simulink model "test_thrust"  (R2024b)
settings: Solver=FixedStepAuto  StartTime=0.0  StopTime=inf  FixedStep=0.01  RelTol=1e-3  EnableMultiTasking=on
libraries: px4Sensorslib x3, px4Peripheralslib x1
settings Model: SimulationMode=external  ExtModeTrigDuration=10  Creator=ArriGE66  LastModifiedBy=xippa
settings SolverCC: PositivePriorityOrder=on
settings OptimizationCC: EnhancedBackFolding=on  PassReuseOutputArgsAs=Individual arguments  ZeroExternalMemoryAtStartup=off  ZeroInternalMemoryAtStartup=off  MaxStackSize=64  OptimizeBlockOrder=speed  DifferentSizesBufferReuse=on  OptimizationCustomize=off  EfficientTunableParamExpr=on
settings DebuggingCC: ParameterTunabilityLossMsg=error
settings HardwareCC: ProdBitPerPointer=32  ProdBitPerSizeT=32  ProdBitPerPtrDiffT=32  ProdLargestAtomicInteger=Long  ProdLargestAtomicFloat=Double  ProdWordSize=32  ProdLongLongMode=on  ProdHWDeviceType=ARM Compatible->ARM Cortex
settings SFSimCC: MATLABDynamicMemAlloc=off  SimTargetLang=C++
settings RTWCC: Description=Embedded Coder  SystemTargetFile=ert.tlc  HardwareBoard=PX4 Cube Orange  TemplateMakefile=ert_default_tmf  Toolchain=GNU Tools for PX4 Autopilots  TargetLang=C++  GPUComputeCapability=3.5
settings CodeAppCC: ForceParamTrailComments=on  IgnoreCustomStorageClasses=off  OperatorAnnotations=on  SimulinkDataObjDesc=on  SFDataObjDesc=on  InsertBlockDesc=on
settings ERTTargetCC: ExtMode=on  ExtModeTransport=3  ExtModeStaticAlloc=on  ExtModeStaticAllocSize=1024  ExtModeMexFile=ext_xcp  ExtModeMexArgs=1 COM10 3000000  ExtModeIntrfLevel=Level2 - Open  InlinedParameterPlacement=Hierarchical  DynamicArrayContainerType=coder::array

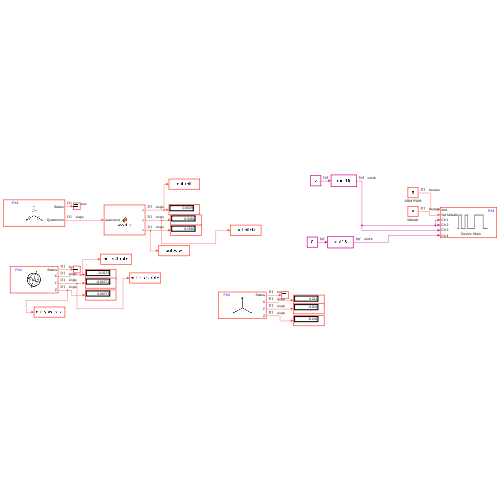
[thumbnail: Simulink's stored preview of the top-level diagram]
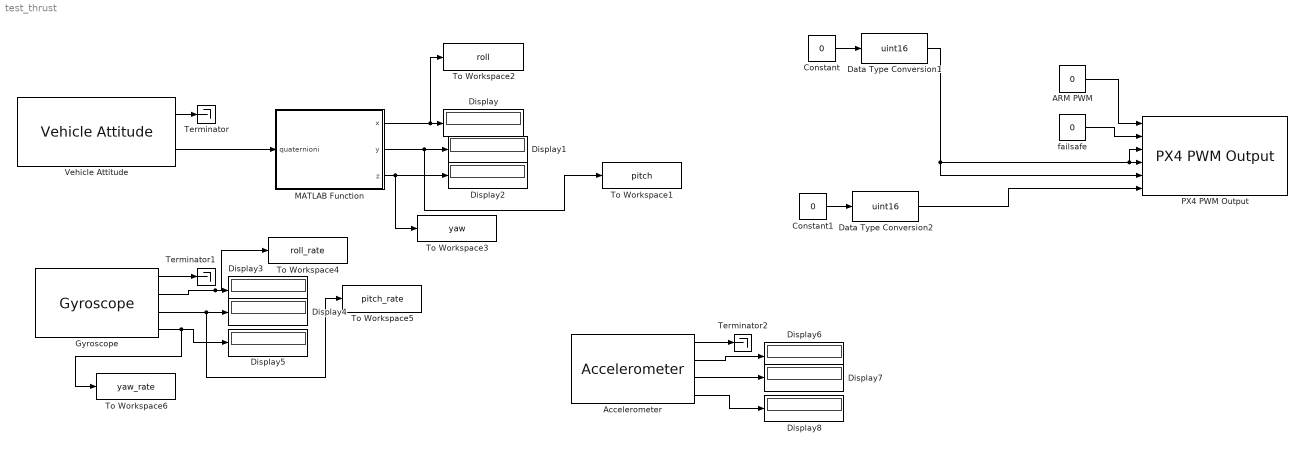
== system test_thrust ==
  ARM PWM : Constant  Value=0  OutDataTypeStr=boolean  SampleTime=1/100
  Accelerometer : px4Sensorslib/Accelerometer  uorbTimeStamp=off  BlockingMode=off  BlockTimeout=1e-3  sampleTime=1/100
  Constant : Constant  Value=0
  Constant1 : Constant  Value=0
  Data Type Conversion1 : DataTypeConversion  OutDataTypeStr=uint16  SaturateOnIntegerOverflow=off  RndMeth=Floor
  Data Type Conversion2 : DataTypeConversion  OutDataTypeStr=uint16  SaturateOnIntegerOverflow=off  RndMeth=Floor
  Display{,1..8} (9 alike) : Display
  Gyroscope : px4Sensorslib/Gyroscope  uorbTimeStamp=off  BlockingMode=off  BlockTimeout=1e-3  sampleTime=1/100
  MATLAB Function : MATLAB Function  TreatAsAtomicUnit=on
  PX4 PWM Output : px4Peripheralslib/PX4 PWM Output  pwmDevice=Main  pwmChannel1_=on  pwmChannel2_=on  pwmChannel3_=on  pwmChannel4_=on  pwmChannel5_=off  pwmChannel6_=off  pwmChannel7_=off  pwmChannel8_=off
  Terminator : Terminator
  Terminator1 : Terminator
  Terminator2 : Terminator
  To Workspace1 : ToWorkspace  VariableName=pitch  SaveFormat=Timeseries  SampleTime=-1
  To Workspace2 : ToWorkspace  VariableName=roll  SaveFormat=Timeseries  SampleTime=-1
  To Workspace3 : ToWorkspace  VariableName=yaw  SaveFormat=Timeseries  SampleTime=-1
  To Workspace4 : ToWorkspace  VariableName=roll_rate  SaveFormat=Timeseries  SampleTime=-1
  To Workspace5 : ToWorkspace  VariableName=pitch_rate  SaveFormat=Timeseries  SampleTime=-1
  To Workspace6 : ToWorkspace  VariableName=yaw_rate  SaveFormat=Timeseries  SampleTime=-1
  Vehicle Attitude : px4Sensorslib/Vehicle Attitude  rollRate=off  pitchRate=off  yawRate=off  quaternion=on  uorbTimeStamp=off  BlockingMode=off  BlockTimeout=0.001  sampleTime=1/100
  failsafe : Constant  Value=0  OutDataTypeStr=boolean  SampleTime=0.01
  wires:
  Vehicle Attitude/2 -> MATLAB Function/1(quaternioni)
  Vehicle Attitude/1 -> Terminator/1
  Data Type Conversion1/1 -> PX4 PWM Output/3, PX4 PWM Output/4, PX4 PWM Output/5
  failsafe/1 -> PX4 PWM Output/2
  Data Type Conversion2/1 -> PX4 PWM Output/6
  ARM PWM/1 -> PX4 PWM Output/1
  Constant/1 -> Data Type Conversion1/1
  Constant1/1 -> Data Type Conversion2/1
  MATLAB Function/3(z) -> To Workspace3/1, Display2/1
  MATLAB Function/2(y) -> To Workspace1/1, Display1/1
  Gyroscope/1 -> Terminator1/1
  Gyroscope/4 -> To Workspace6/1, Display5/1
  Gyroscope/3 -> To Workspace5/1, Display4/1
  Gyroscope/2 -> To Workspace4/1, Display3/1
  Accelerometer/4 -> Display8/1
  Accelerometer/1 -> Terminator2/1
  Accelerometer/3 -> Display7/1
  Accelerometer/2 -> Display6/1
  MATLAB Function/1(x) -> To Workspace2/1, Display/1

== matlab function test_thrust/MATLAB Function ==
  data: x output; quaternioni input; y output; z output
function [x, y, z] = assetto(quaternioni)
    % Estrazione dei componenti del quaternione
    qw = quaternioni(1);
    qx = quaternioni(2);
    qy = quaternioni(3);
    qz = quaternioni(4);

    % Calcolo degli angoli di Eulero manualmente
    x = atan2(2*(qw*qx + qy*qz), 1 - 2*(qx^2 + qy^2)); % roll
    y = asin(2*(qw*qy - qz*qx));                          % Pitch
    z = atan2(2*(qw*qz + qx*qy), 1 - 2*(qy^2 + qz^2));   % yaw
end
